simulink library "MdlLib_ProcessOutput"  (R2019a)
settings: Solver=VariableStepAuto  StartTime=0.0  StopTime=10.0  RelTol=1e-3
values from neighbouring files (symbols this model uses):
  omegabar = interp1(Lin_points.V,Lin_points.RSpeed,Vbar,'spline')    [testCtrl.m]
settings Model: Creator=ditt_aj  LastModifiedBy=ditt_aj

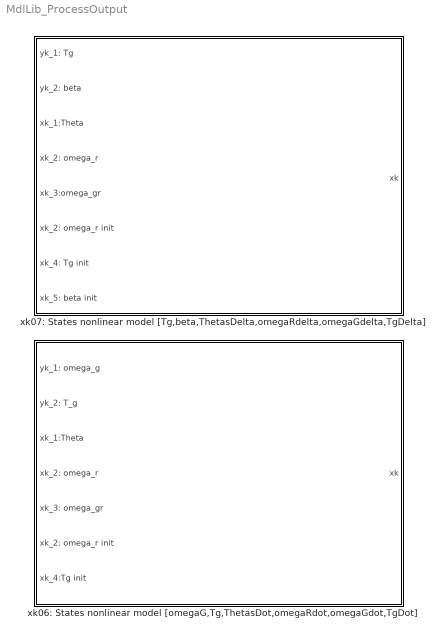
== system MdlLib_ProcessOutput ==
  xk06: States nonlinear model [omegaG,Tg,ThetasDot,omegaRdot,omegaGdot,TgDot] : Subsystem
  xk07: States nonlinear model [Tg,beta,ThetasDelta,omegaRdelta,omegaGdelta,TgDelta] : Subsystem

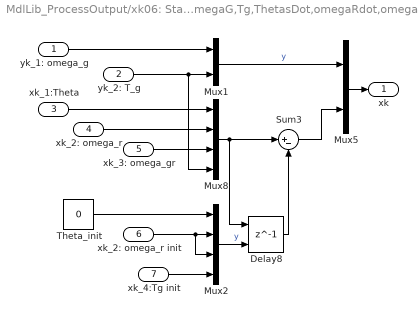
== system MdlLib_ProcessOutput/xk06: States nonlinear model [omegaG,Tg,ThetasDot,omegaRdot,omegaGdot,TgDot] ==
  yk_1: omega_g : Inport
  yk_2: T_g : Inport  Port=2
  xk_1:Theta : Inport  Port=3
  xk_2: omega_r : Inport  Port=4
  "xk_3: omega_gr " : Inport  Port=5
  xk_2: omega_r init : Inport  Port=6
  xk_4:Tg init : Inport  Port=7
  Delay8 : Delay  DelayLength=1  InitialConditionSource=Input port  InitialCondition=[0,omegabar]
      settings: InputPortMap=u0,p4
  Mux1 : Mux  Inputs=2
  Mux2 : Mux
  Mux5 : Mux  Inputs=2
  Mux8 : Mux
  Sum3 : Sum  Inputs=|+-
  Theta_init : Constant  Value=0
  xk : Outport
  wires:
  Sum3/1 -> Mux5/2
  yk_1: omega_g/1 -> Mux1/1
  Delay8/1 -> Sum3/2
  yk_2: T_g/1 -> Mux8/4, Mux1/2
  Mux8/1 -> Delay8/1, Sum3/1
  Mux1/1 -> Mux5/1  "y"
  Mux2/1 -> Delay8/2  "y"
  Mux5/1 -> xk/1
  "xk_3: omega_gr "/1 -> Mux8/3
  xk_2: omega_r/1 -> Mux8/2
  xk_1:Theta/1 -> Mux8/1
  Theta_init/1 -> Mux2/1
  xk_2: omega_r init/1 -> Mux2/3, Mux2/2
  xk_4:Tg init/1 -> Mux2/4

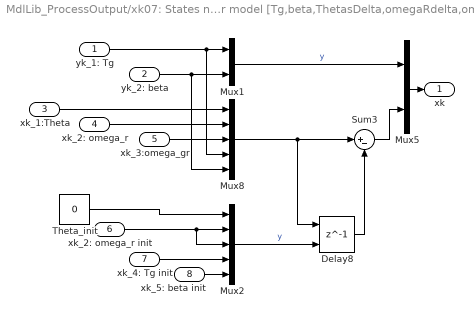
== system MdlLib_ProcessOutput/xk07: States nonlinear model [Tg,beta,ThetasDelta,omegaRdelta,omegaGdelta,TgDelta] ==
  yk_1: Tg : Inport
  yk_2: beta : Inport  Port=2
  xk_1:Theta : Inport  Port=3
  xk_2: omega_r : Inport  Port=4
  "xk_3:omega_gr " : Inport  Port=5
  xk_2: omega_r init : Inport  Port=6
  xk_4: Tg init : Inport  Port=7
  xk_5: beta init : Inport  Port=8
  Delay8 : Delay  DelayLength=1  InitialConditionSource=Input port  InitialCondition=[0,omegabar]
      settings: InputPortMap=u0,p4
  Mux1 : Mux  Inputs=2
  Mux2 : Mux  Inputs=5
  Mux5 : Mux  Inputs=2
  Mux8 : Mux  Inputs=5
  Sum3 : Sum  Inputs=|+-
  Theta_init : Constant  Value=0
  xk : Outport
  wires:
  Sum3/1 -> Mux5/2
  yk_1: Tg/1 -> Mux8/4, Mux1/1
  Delay8/1 -> Sum3/2
  yk_2: beta/1 -> Mux8/5, Mux1/2
  Mux8/1 -> Delay8/1, Sum3/1
  Mux1/1 -> Mux5/1  "y"
  Mux2/1 -> Delay8/2  "y"
  Mux5/1 -> xk/1
  "xk_3:omega_gr "/1 -> Mux8/3
  xk_2: omega_r/1 -> Mux8/2
  xk_1:Theta/1 -> Mux8/1
  xk_5: beta init/1 -> Mux2/5
  Theta_init/1 -> Mux2/1
  xk_2: omega_r init/1 -> Mux2/3, Mux2/2
  xk_4: Tg init/1 -> Mux2/4
